simulink model "PIDoven"  (R2022b)
settings: Solver=ode23  StartTime=0.0  StopTime=80000  FixedStep=1e-6  RelTol=1e-19  AbsTol=1e-19
settings Model: Creator=svens  LastModifiedBy=saraa
settings SolverCC: ZeroCrossAlgorithm=Adaptive
settings DebuggingCC: IgnoredZcDiagnostic=none

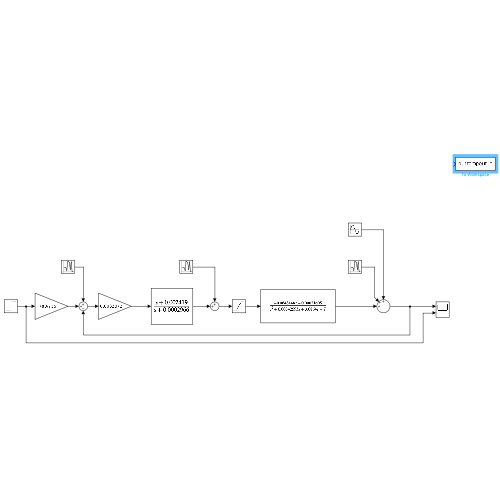
[thumbnail: Simulink's stored preview of the top-level diagram]
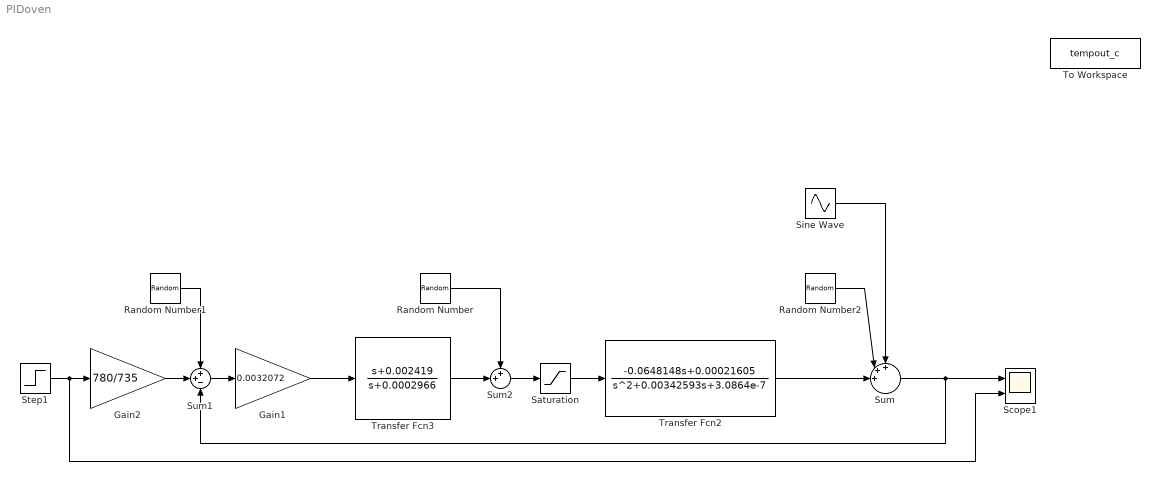
== system PIDoven ==
  Gain1 : Gain  Gain=0.0032072
  Gain2 : Gain  Gain=780/735
  Random Number : RandomNumber  Variance=20  SampleTime=0.1
  Random Number1 : RandomNumber  Variance=20  SampleTime=0.1
  Random Number2 : RandomNumber  Variance=20  SampleTime=7800
  Saturation : Saturate  UpperLimit=2  LowerLimit=0  LinearizeAsGain=off
  Scope1 : Scope  NumInputPorts=2
  Sine Wave : Sin  Amplitude=6  Bias=25  Frequency=7.2e-5  SampleTime=0
  Step1 : Step  After=780  SampleTime=0
  Sum : Sum  Inputs=+++||
  Sum1 : Sum  Inputs=++-
  Sum2 : Sum  Inputs=++|
  To Workspace : ToWorkspace  VariableName=tempout_c  SaveFormat=Timeseries  SampleTime=-1
  Transfer Fcn2 : TransferFcn  Numerator=[-0.0648148 0.00021605]  Denominator=[1 0.00342593 3.0864e-7]
  Transfer Fcn3 : TransferFcn  Numerator=[1 0.002419]  Denominator=[1 0.0002966]
  wires:
  Gain1/1 -> Transfer Fcn3/1
  Sum1/1 -> Gain1/1
  Transfer Fcn3/1 -> Sum2/2
  Transfer Fcn2/1 -> Sum/3
  Sum2/1 -> Saturation/1
  Random Number/1 -> Sum2/1
  Random Number1/1 -> Sum1/1
  Saturation/1 -> Transfer Fcn2/1
  Sine Wave/1 -> Sum/1
  Random Number2/1 -> Sum/2
  Step1/1 -> Scope1/2, Gain2/1
  Gain2/1 -> Sum1/2
  Sum/1 -> Sum1/3, Scope1/1
